simulink model "sschdlexResonantLLCConverterModel"  (R2026a)
settings: Solver=FixedStepDiscrete  StopTime=1e-3
PreLoadFcn:
  | Vdc = 340;
  | Vbus_nominal = 450;
  | Vbus_ripple = 10;
  | busRippleFrequency = 100;
  | Vout_nominal = 54;
  | Pout = 100;
  | Cr = 1.2089e-8;
  | Lr = 1.6226e-4;
  | Lm = 2.3e-3;
  | TR = 4.3269;
  | transformerCoupling = 0.99;
  | Cout = 3.0237e-5;
  | Vf = 0.6;
  | 
  | F_FPGA = 50e6;
  | ts_FPGA_clk  = 1/F_FPGA;
  | ts_cpu= 5e-5;
  | fsw = 100e3;
  | Tbase = ts_FPGA_clk;
  | ts_FPGA_mdl = ts_FPGA_clk;
  | Tdata= ts_FPGA_mdl;
  | 
  | Ts_CAN_Tx = 1e-2;
  | switchType =2 ;
PostLoadFcn:
  | FPGASubsystem_HDLSubsystem_LLCConverter_SolverConfiguration_Gs = Simulink.Parameter;
  | FPGASubsystem_HDLSubsystem_LLCConverter_SolverConfiguration_Gs.Value = 1;
  | FPGASubsystem_HDLSubsystem_LLCConverter_SolverConfiguration_s = Simulink.Parameter;
  | FPGASubsystem_HDLSubsystem_LLCConverter_SolverConfiguration_s.Value = 1;
libraries: SimscapeFPGAHIL_lib x8, ee_lib x6, fl_lib x5, nesl_utility x3, hdlsllib x2
settings Model: DataTypeOverride=Off  Creator=The MathWorks, Inc.  LastModifiedBy=The MathWorks, Inc.
settings OptimizationCC: ConditionallyExecuteInputs=off  InheritOutputTypeSmallerThanSingle=on
settings DebuggingCC: ArtificialAlgebraicLoopMsg=error  SingleTaskRateTransMsg=error
settings HardwareCC: ProdHWDeviceType=ASIC/FPGA->ASIC/FPGA  TargetBitPerLong=64.0  TargetBitPerPointer=64.0  TargetBitPerSizeT=64.0  TargetBitPerPtrDiffT=64.0  TargetLongLongMode=on  TargetIntDivRoundTo=Zero  TargetEndianess=LittleEndian  TargetWordSize=64.0  TargetHWDeviceType=Custom Processor->MATLAB Host Computer  ProdEqTarget=off
settings SimscapeCC: SimscapeNominalValues="[{\"value\":\"1\",\"unit\":\"A\"},{\"value\":\"1\",\"unit\":\"bar\"},{\"value\":\"1\",\"unit\":\"cm^2\"},{\"value\":\"1\",\"unit\":\"cm^3/s\"},{\"value\":\"1\",\"unit\":\"kJ/kg\"},{\"value\":\"1\",\"unit\":\"kW\"},{\"value\":\"1\",\"unit\":\"l\"},{\"value\":\"1\",\"unit\":\"N\"},{\"value\":\"1\",\"unit\":\"N*m\"},{\"value\":\"1\",\"unit\":\"V\"}]"  SimscapeLogType=none  SimscapeLogDataHistory=5000.0

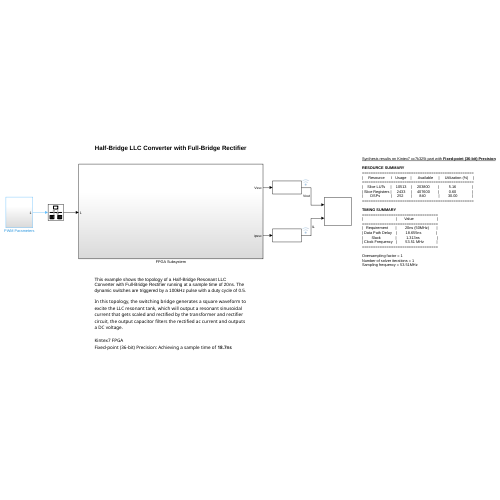
[thumbnail: Simulink's stored preview of the top-level diagram]
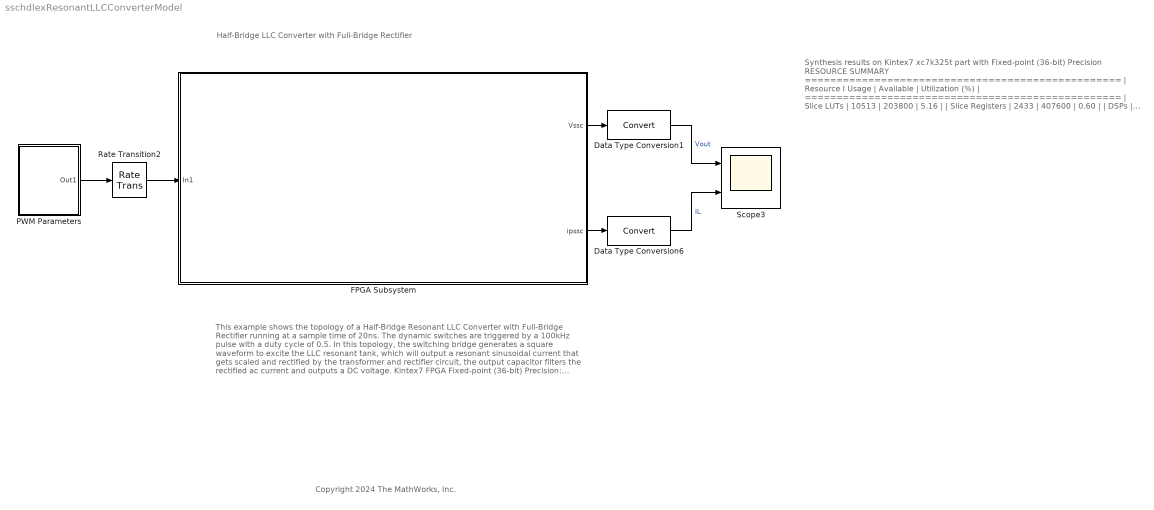
== system sschdlexResonantLLCConverterModel ==
  note: This example shows the topology of a Half-Bridge Resonant LLC Converter with Full-Bridge Rectifier running at a sample time of 20ns. The dynamic switches are triggered by a 100kHz pulse with a duty cycle of 0.5.
      |
      | In this topology, the switching bridge generates a square waveform to excite the LLC resonant tank, which will output a resonant sinusoidal current that gets scaled and rectified by the transformer and rectifier circuit, the output capacitor filters the rectified ac current and outputs a DC voltage.
      |
      | Kintex7 FPGA
      | Fixed-point (36-bit) Precision: Achieving a sample time of 18.7ns
  note: Half-Bridge LLC Converter with Full-Bridge Rectifier
  note: Synthesis results on Kintex7 xc7k325t part with Fixed-point (36-bit) Precision
      |
      | RESOURCE SUMMARY
      | ==================================================
      | | Resource I Usage | Available | Utilization (%) |
      | ==================================================
      | | Slice LUTs | 10513 | 203800 | 5.16 |
      | | Slice Registers | 2433 | 407600 | 0.60 |
      | | DSPs | 252 | 840 | 30.00 |
      | ==================================================
      |
      | TIMING SUMMARY
      | ==================================
      | | | Value |
      | ==================================
      | | Requirement | 20ns (50MHz) |
      | | Data Path Delay | 18.655ns |
      | | Slack | 1.313ns |
      | | Clock Frequency | 53.51 MHz |
      | ==================================
      |
      | Oversampling factor = 1
      | Number of solver iterations = 1
      | Sampling frequency = 53.51MHz
  note: Copyright 2024 The MathWorks, Inc.
  Data Type Conversion1 : DataTypeConversion  SaturateOnIntegerOverflow=off  RndMeth=Floor
  Data Type Conversion6 : DataTypeConversion  SaturateOnIntegerOverflow=off  RndMeth=Floor
  FPGA Subsystem : Subsystem
  PWM Parameters : Subsystem
  Rate Transition2 : RateTransition  OutPortSampleTime=ts_FPGA_clk
  Scope3 : Scope  NumInputPorts=2
      settings: ActiveDisplayYMinimum=-10.52759  ActiveDisplayYMaximum=94.7483
  wires:
  Data Type Conversion1/1 -> Scope3/1  "Vout"
  Data Type Conversion6/1 -> Scope3/2  "IL"
  PWM Parameters/1(Out1) -> Rate Transition2/1
  Rate Transition2/1 -> FPGA Subsystem/1(In1)
  FPGA Subsystem/1(Vssc) -> Data Type Conversion1/1
  FPGA Subsystem/2(ipssc) -> Data Type Conversion6/1

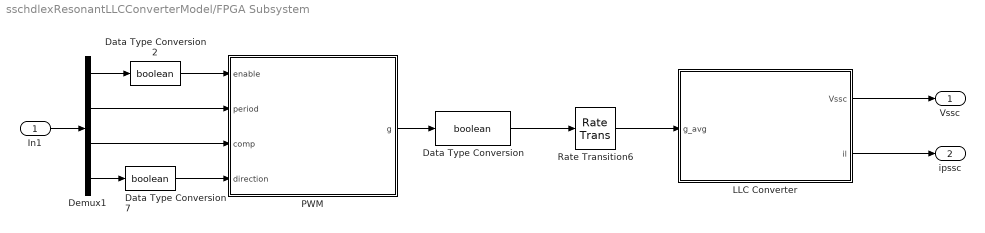
== system sschdlexResonantLLCConverterModel/FPGA Subsystem ==
  In1 : Inport
  Data Type Conversion : DataTypeConversion  OutDataTypeStr=boolean  SaturateOnIntegerOverflow=off  RndMeth=Floor
  Data Type Conversion2 : DataTypeConversion  OutDataTypeStr=boolean  SaturateOnIntegerOverflow=off  RndMeth=Floor
  Data Type Conversion7 : DataTypeConversion  OutDataTypeStr=boolean  SaturateOnIntegerOverflow=off  RndMeth=Floor
  Demux1 : Demux
  LLC Converter : Subsystem
  PWM : Subsystem
  Rate Transition6 : RateTransition
  Vssc : Outport
  ipssc : Outport  Port=2
  wires:
  Demux1/4 -> Data Type Conversion7/1
  Data Type Conversion2/1 -> PWM/1(enable)
  In1/1 -> Demux1/1
  Demux1/1 -> Data Type Conversion2/1
  PWM/1(g) -> Data Type Conversion/1
  Data Type Conversion7/1 -> PWM/4(direction)
  Demux1/3 -> PWM/3(comp)
  Demux1/2 -> PWM/2(period)
  LLC Converter/1(Vssc) -> Vssc/1
  LLC Converter/2(il) -> ipssc/1
  Data Type Conversion/1 -> Rate Transition6/1
  Rate Transition6/1 -> LLC Converter/1(g_avg)

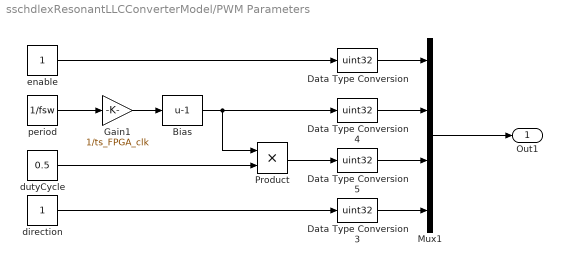
== system sschdlexResonantLLCConverterModel/PWM Parameters ==
  Bias : Bias  Bias=-1  SaturateOnIntegerOverflow=off
  Data Type Conversion{,3..5} (4 alike) : DataTypeConversion  OutDataTypeStr=uint32  SaturateOnIntegerOverflow=off  RndMeth=Floor
  Gain1 : Gain  Gain=1/ts_FPGA_clk
  Mux1 : Mux
  Product : Product
  direction : Constant  SampleTime=ts_cpu
  dutyCycle : Constant  Value=0.5  SampleTime=ts_cpu
  enable : Constant  SampleTime=ts_cpu
  period : Constant  Value=1/fsw  SampleTime=ts_cpu
  Out1 : Outport
  wires:
  Mux1/1 -> Out1/1
  Data Type Conversion/1 -> Mux1/1
  dutyCycle/1 -> Product/2
  Product/1 -> Data Type Conversion5/1
  Gain1/1 -> Bias/1
  Data Type Conversion4/1 -> Mux1/2
  Data Type Conversion3/1 -> Mux1/4
  Data Type Conversion5/1 -> Mux1/3
  period/1 -> Gain1/1
  Bias/1 -> Product/1, Data Type Conversion4/1
  direction/1 -> Data Type Conversion3/1
  enable/1 -> Data Type Conversion/1

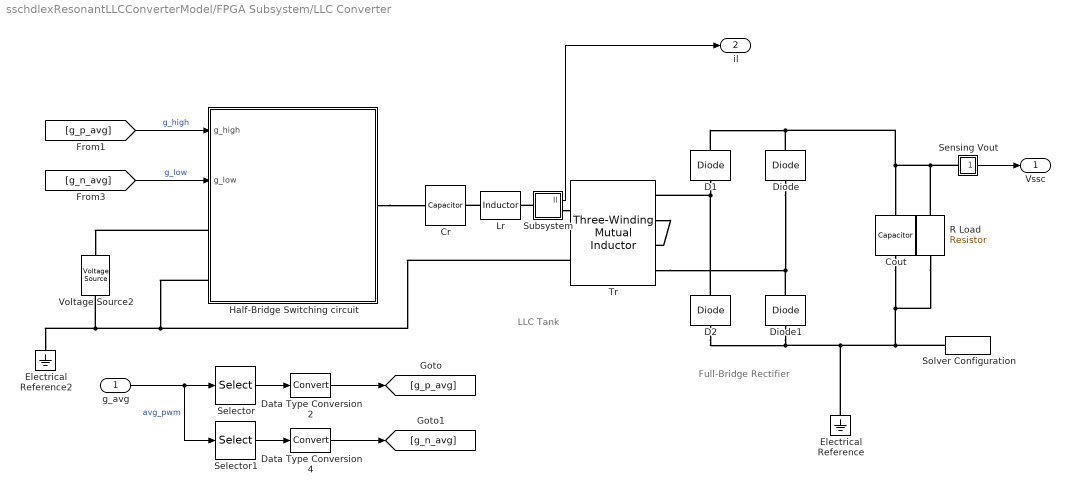
== system sschdlexResonantLLCConverterModel/FPGA Subsystem/LLC Converter ==
  note: LLC Tank
  note: Full-Bridge Rectifier
  g_avg : Inport
  " Half-Bridge Switching circuit" : Subsystem  VariantControl=HB
  Cout : ee_lib/Passive/Capacitor  cap_option=ee.enum.passive.capacitor.capOption.const  c=Cout F  Cvec=[ 1e-5 1e-6 ] F  Vvec=[ 0 10 ] V  CV_table_symmetry=1  f_vec=[1, 10] kHz  DFext_vec=[.8, 1.2]  enable_C_tol=0  averaging_period=0 s  C_tol=5  tol_distribution=1  nSigma=4  r=1e-6 Ohm  g=0 1/Ohm  enable_operating_limits=0  operating_limit_action=2  max_working_voltage_range=[ -25 25 ] V  power_rating=1 W  maxTemperature=85 degC  thermalEnable=false  thermalMass=1 J/K  i_specify=off  i_priority=None  i=0 A  i_nominal_specify=off  i_nominal_value=1  i_nominal_unit=A  v_specify=off  v_priority=None  v=0 V  v_nominal_specify=off  v_nominal_value=1  v_nominal_unit=V  vc_specify=on  vc_priority=High  vc=0 V  vc_nominal_specify=off  vc_nominal_value=1  vc_nominal_unit=V  T_specify=off  T_priority=None  T=298.15 K  T_nominal_specify=off  T_nominal_value=1  T_nominal_unit=K
  Cr : ee_lib/Passive/Capacitor  cap_option=ee.enum.passive.capacitor.capOption.const  c=Cr F  Cvec=[ 1e-5 1e-6 ] F  Vvec=[ 0 10 ] V  CV_table_symmetry=1  f_vec=[1, 10] kHz  DFext_vec=[.8, 1.2]  enable_C_tol=0  averaging_period=0 s  C_tol=5  tol_distribution=1  nSigma=4  r=1e-6 Ohm  g=1e-6 1/Ohm  enable_operating_limits=0  operating_limit_action=2  max_working_voltage_range=[ -25 25 ] V  power_rating=1 W  maxTemperature=85 degC  thermalEnable=false  thermalMass=1 J/K  i_specify=off  i_priority=None  i=0 A  i_nominal_specify=off  i_nominal_value=1  i_nominal_unit=A  v_specify=off  v_priority=None  v=0 V  v_nominal_specify=off  v_nominal_value=1  v_nominal_unit=V  vc_specify=on  vc_priority=High  vc=0 V  vc_nominal_specify=off  vc_nominal_value=1  vc_nominal_unit=V  T_specify=off  T_priority=None  T=298.15 K  T_nominal_specify=off  T_nominal_value=1  T_nominal_unit=K
  D1 : SimscapeFPGAHIL_lib/Dynamic Switch Models/Diode  Vf=0.6  Gs=FPGASubsystem_HDLSubsystem_LLCConverter_SolverConfiguration_Gs  s=FPGASubsystem_HDLSubsystem_LLCConverter_SolverConfiguration_s
  D2 : SimscapeFPGAHIL_lib/Dynamic Switch Models/Diode  Vf=0.6  Gs=FPGASubsystem_HDLSubsystem_LLCConverter_SolverConfiguration_Gs  s=FPGASubsystem_HDLSubsystem_LLCConverter_SolverConfiguration_s
  Data Type Conversion2 : DataTypeConversion  SaturateOnIntegerOverflow=off  RndMeth=Floor
  Data Type Conversion4 : DataTypeConversion  SaturateOnIntegerOverflow=off  RndMeth=Floor
  Diode : SimscapeFPGAHIL_lib/Dynamic Switch Models/Diode  Vf=0.6  Gs=FPGASubsystem_HDLSubsystem_LLCConverter_SolverConfiguration_Gs  s=FPGASubsystem_HDLSubsystem_LLCConverter_SolverConfiguration_s
  Diode1 : SimscapeFPGAHIL_lib/Dynamic Switch Models/Diode  Vf=0.6  Gs=FPGASubsystem_HDLSubsystem_LLCConverter_SolverConfiguration_Gs  s=FPGASubsystem_HDLSubsystem_LLCConverter_SolverConfiguration_s
  Electrical Reference : fl_lib/Electrical/Electrical Elements/Electrical Reference
  Electrical Reference2 : fl_lib/Electrical/Electrical Elements/Electrical Reference
  Lr : ee_lib/Passive/Inductor  l=Lr H  enable_L_tol=0  L_tol=20  tol_distribution=1  nSigma=4  r=0 Ohm  g=1e-9 1/Ohm  enable_operating_limits=0  operating_limit_action=2  max_working_current=1 A  power_rating=1 W  i_L_specify=on  i_L_priority=High  i_L=0 A  i_L_nominal_specify=off  i_L_nominal_value=1  i_L_nominal_unit=A
  R Load : ee_lib/Passive/Resistor  R=Vout_nominal^2/Pout Ohm  enable_R_tol=0  R_tol=5  tol_distribution=1  nSigma=4  enable_operating_limits=0  operating_limit_action=2  power_rating=1 W  max_working_voltage=100 V  noise_mode=0  Tdevice=25 degC  sample_time=0.001 s  repeatability=1  user_seed=0  auto_seed=2715962282  power_derating_T1=70 degC  power_derating_T2=155 degC  operating_temperature_range_vec=[-50, 150] degC  alpha=3.93e-3 1/K  Tmeas=25 degC  thermal_mass=100 J/K  temperature_specify=off  temperature_priority=High  temperature=298.15 K  temperature_nominal_specify=off  temperature_nominal_value=1  temperature_nominal_unit=K
  Selector : Selector  InputPortWidth=2  IndexOptions=Index vector (dialog)  Indices=1  OutputSizes=1
  Selector1 : Selector  InputPortWidth=2  IndexOptions=Index vector (dialog)  Indices=2  OutputSizes=1
  Sensing Vout : Subsystem
      mask Display: disp('v')
  Solver Configuration : nesl_utility/Solver Configuration  PhysicalDomain=network_engine_domain  SubClassName=solver  LeftPortType=input  RightPortType=generic  Tones=[]  Harmonics=[]  SimulateNoise=off  Profile=off  UseLocalSampling=off  EnableSwitchedLinearOptims=on  FrequencyDomain=off  UseCCode=off  RelTol=0.001  AbsTol=1e-06  MinStep=1e-09  ToWorkspace=off  RevertToSquareIcSolve=off  NumHomotopyIterations=100  PhasorMode=off  PhasorModeNumHarmonics=1  ConsistencySolver=NEWTON_FTOL  CanonicalOrdering=UNORDERED  OptimizeIntermediates=UNOPTIMIZED  IndexReductionMethod=DerivativeReplacement  DoDC=off  ResidualTolerance=1e-09  ConsistencyTolSource=GLOBAL  ConsistencyAbsTol=0.001  ConsistencyRelTol=0.001  ConsistencyTolFactor=0.001  UseLocalSolver=on  LocalSolverChoice=NE_BACKWARD_EULER_ADVANCER  ResolveIndetEquations=on  FunctionEvalNumThread=1  LocalSolverSampleTime=ts_FPGA_mdl  DoFixedCost=off  MaxNonlinIter=2  MaxModeIter=2  ComputeImpulses=off  ImpulseIterations=2  LinearAlgebra=auto  LinearAlgebraNumThread=0  EquationFormulation=NE_TIME_EF  DelaysMemoryBudget=1024  AutomaticFiltering=on  FilteringTimeConstant=0.001  PartitionStorageMethod=AS_NEEDED  PartitionMemoryBudget=1024  PartitionMethod=FAST  MultibodyUseLocalSolver=off  MultibodyLocalSolverChoice=ODE1  MultibodyLocalSolverSampleTime=0.001
  Subsystem : Subsystem
  Tr : ee_lib/Passive/Transformers/Three-Winding Mutual Inductor  L1=Lm/transformerCoupling^2 H  L2=Lm/TR^2 H  L3=Lm/TR^2 H  perfectCoupling=false  K12=transformerCoupling  K13=transformerCoupling  K23=transformerCoupling  i1_specify=off  i1_priority=None  i1=0 A  i1_nominal_specify=off  i1_nominal_value=1  i1_nominal_unit=A  i2_specify=on  i2_priority=High  i2=0 A  i2_nominal_specify=off  i2_nominal_value=1  i2_nominal_unit=A  i3_specify=off  i3_priority=None  i3=0 A  i3_nominal_specify=off  i3_nominal_value=1  i3_nominal_unit=A
  Voltage Source2 : ee_lib/Sources/Voltage Source  dc_voltage=Vdc V  ac_voltage=0 V  ac_shift=0 rad  ac_frequency=60 Hz  noise_mode=ee.enum.sources.noise.Disabled  PSD=0 V^2/Hz  sample_time=1e-3 s  repeatability=ee.enum.sources.repeatability.NotRepeatable  user_seed=0  auto_seed=781027040  i_specify=off  i_priority=None  i=0 A  i_nominal_specify=off  i_nominal_value=1  i_nominal_unit=A  v_specify=off  v_priority=None  v=0 V  v_nominal_specify=off  v_nominal_value=1  v_nominal_unit=V
  Vssc : Outport
  il : Outport  Port=2
  wires:
  Data Type Conversion4/1 -> [g_n_avg]
  Data Type Conversion2/1 -> [g_p_avg]
  Selector/1 -> Data Type Conversion2/1
  Selector1/1 -> Data Type Conversion4/1
  g_avg/1 -> Selector/1, Selector1/1  "avg_pwm"
  [g_p_avg] -> " Half-Bridge Switching circuit"/1(g_high)  "g_high"
  [g_n_avg] -> " Half-Bridge Switching circuit"/2(g_low)  "g_low"
  Subsystem/1(Il) -> il/1
  Sensing Vout/1(v) -> Vssc/1
  connections:
  Tr/LConn2 -- " Half-Bridge Switching circuit"/LConn2 -- Electrical Reference2/LConn1 -- Voltage Source2/RConn1
  " Half-Bridge Switching circuit"/LConn1 -- Voltage Source2/LConn1
  Lr/LConn1 -- Cr/RConn1
  Subsystem/RConn1 -- Tr/LConn1
  " Half-Bridge Switching circuit"/RConn1 -- Cr/LConn1
  Subsystem/LConn1 -- Lr/RConn1
  Tr/RConn2 -- Tr/RConn3
  Tr/RConn4 -- Diode/LConn1 -- Diode1/RConn1
  D1/LConn1 -- Tr/RConn1 -- D2/RConn1
  Sensing Vout/LConn1 -- R Load/LConn1 -- D1/RConn1 -- Diode/RConn1 -- Cout/LConn1
  Cout/RConn1 -- Solver Configuration/RConn1 -- Electrical Reference/LConn1 -- D2/LConn1 -- Diode1/LConn1 -- R Load/RConn1

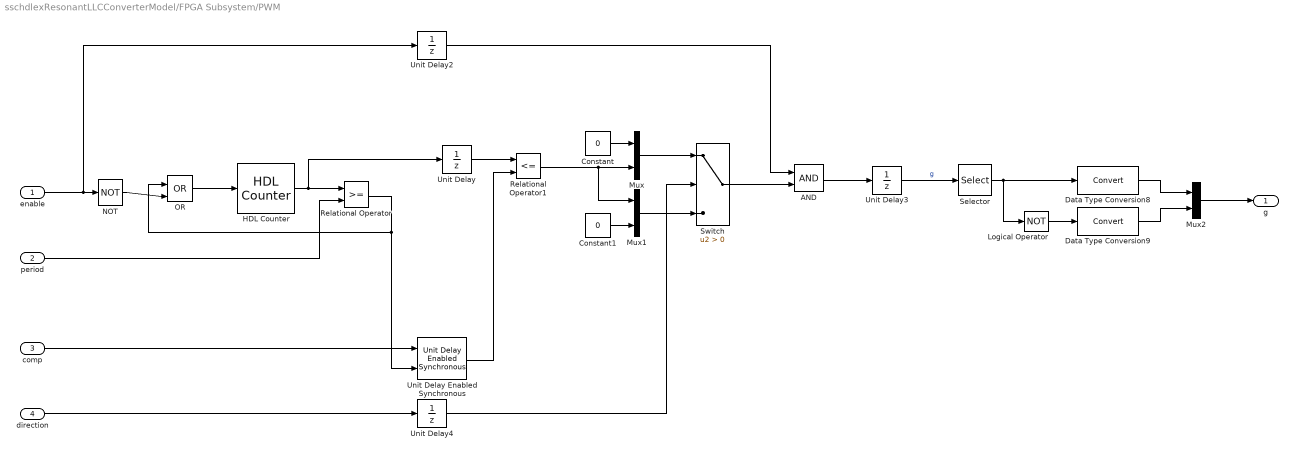
== system sschdlexResonantLLCConverterModel/FPGA Subsystem/PWM ==
  enable : Inport
  period : Inport  Port=2
  comp : Inport  Port=3
  direction : Inport  Port=4
  AND : Logic  AllPortsSameDT=off  OutDataTypeStr=boolean
  Constant : Constant  Value=0  OutDataTypeStr=boolean  SampleTime=-1
  Constant1 : Constant  Value=0  OutDataTypeStr=boolean  SampleTime=-1
  Data Type Conversion8 : DataTypeConversion  SaturateOnIntegerOverflow=off  RndMeth=Floor
  Data Type Conversion9 : DataTypeConversion  SaturateOnIntegerOverflow=off  RndMeth=Floor
  HDL Counter : hdlsllib/Sources/HDL Counter  CountType=Free running  CountInit=0  CountStep=1  CountMax=25  CountFromType=Initial value  CountFrom=0  CountResetPort=on  CountLoadPort=off  CountEnbPort=off  CountDirPort=off  CountHitOutputPort=off  CountDataType=Unsigned  CountWordLen=32  CountFracLen=0  CountSampTime=1
  Logical Operator : Logic  Operator=NOT  AllPortsSameDT=off  OutDataTypeStr=boolean
  Mux : Mux  Inputs=2
  Mux1 : Mux  Inputs=2
  Mux2 : Mux  Inputs=2
  NOT : Logic  Operator=NOT  AllPortsSameDT=off  OutDataTypeStr=boolean
  OR : Logic  Operator=OR  IconShape=distinctive  AllPortsSameDT=off  OutDataTypeStr=boolean
  Relational Operator : RelationalOperator  OutDataTypeStr=boolean  RndMeth=Simplest  InputSameDT=off
  Relational Operator1 : RelationalOperator  Operator=<=  OutDataTypeStr=boolean  RndMeth=Simplest  InputSameDT=off
  Selector : Selector  InputPortWidth=2  IndexOptions=Index vector (dialog)  Indices=[2]  OutputSizes=1
  Switch : Switch  Criteria=u2 > Threshold  SaturateOnIntegerOverflow=off  InputSameDT=off
  Unit Delay{,2..4} (4 alike) : UnitDelay  SampleTime=-1
  Unit Delay Enabled Synchronous : hdlsllib/Discrete/Unit Delay Enabled Synchronous  InitialCondition=0.0  SampleTime=-1
  g : Outport
  wires:
  comp/1 -> Unit Delay Enabled Synchronous/1
  Unit Delay3/1 -> Selector/1  "g"
  period/1 -> Relational Operator/2
  Switch/1 -> AND/2
  Unit Delay/1 -> Relational Operator1/1
  direction/1 -> Unit Delay4/1
  AND/1 -> Unit Delay3/1
  Mux/1 -> Switch/1
  Constant1/1 -> Mux1/2
  Unit Delay2/1 -> AND/1
  Mux1/1 -> Switch/3
  Constant/1 -> Mux/1
  Relational Operator/1 -> OR/1, Unit Delay Enabled Synchronous/2
  enable/1 -> NOT/1, Unit Delay2/1
  HDL Counter/1 -> Relational Operator/1, Unit Delay/1
  Unit Delay4/1 -> Switch/2
  Unit Delay Enabled Synchronous/1 -> Relational Operator1/2
  OR/1 -> HDL Counter/1
  Relational Operator1/1 -> Mux/2, Mux1/1
  NOT/1 -> OR/2
  Data Type Conversion9/1 -> Mux2/2
  Data Type Conversion8/1 -> Mux2/1
  Logical Operator/1 -> Data Type Conversion9/1
  Selector/1 -> Logical Operator/1, Data Type Conversion8/1
  Mux2/1 -> g/1

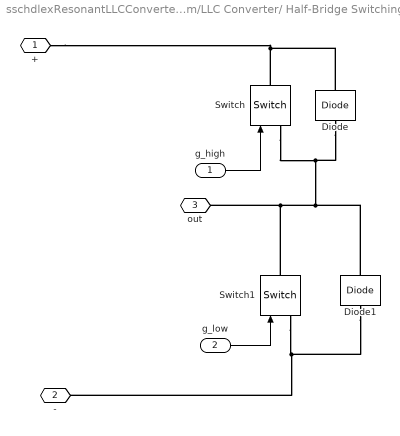
== system sschdlexResonantLLCConverterModel/FPGA Subsystem/LLC Converter/ Half-Bridge Switching circuit ==
  g_high : Inport
  g_low : Inport  Port=2
  Diode : SimscapeFPGAHIL_lib/Dynamic Switch Models/Diode  Vf=0.6  Gs=FPGASubsystem_HDLSubsystem_LLCConverter_SolverConfiguration_Gs  s=FPGASubsystem_HDLSubsystem_LLCConverter_SolverConfiguration_s
  Diode1 : SimscapeFPGAHIL_lib/Dynamic Switch Models/Diode  Vf=0.6  Gs=FPGASubsystem_HDLSubsystem_LLCConverter_SolverConfiguration_Gs  s=FPGASubsystem_HDLSubsystem_LLCConverter_SolverConfiguration_s
  Switch : SimscapeFPGAHIL_lib/Dynamic Switch Models/Switch  device_type=Switch  threshold=0.5  Gs=FPGASubsystem_HDLSubsystem_LLCConverter_SolverConfiguration_Gs  s=FPGASubsystem_HDLSubsystem_LLCConverter_SolverConfiguration_s
  Switch1 : SimscapeFPGAHIL_lib/Dynamic Switch Models/Switch  device_type=Switch  threshold=0.5  Gs=FPGASubsystem_HDLSubsystem_LLCConverter_SolverConfiguration_Gs  s=FPGASubsystem_HDLSubsystem_LLCConverter_SolverConfiguration_s
  + : PMIOPort  Side=Left
  - : PMIOPort  Port=2  Side=Left
  out : PMIOPort  Port=3  Side=Right
  wires:
  g_high/1 -> Switch/1
  g_low/1 -> Switch1/1
  connections:
  +/RConn1 -- Diode/RConn1 -- Switch/RConn1
  Diode1/LConn1 -- Switch1/LConn1 -- -/RConn1
  Diode/LConn1 -- Switch/LConn1 -- out/RConn1 -- Switch1/RConn1 -- Diode1/RConn1

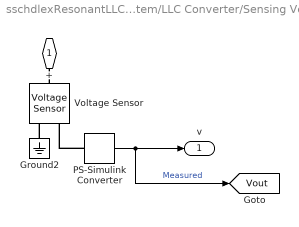
== system sschdlexResonantLLCConverterModel/FPGA Subsystem/LLC Converter/Sensing Vout ==
  Ground2 : fl_lib/Electrical/Electrical Elements/Electrical Reference
  PS-Simulink Converter : nesl_utility/PS-Simulink Converter  PhysicalDomain=network_engine_domain  SubClassName=ps_output  LeftPortType=input  RightPortType=output  PseudoPeriodic=off  Frequencies=[]  VectorFormat=1-D array  Unit=1  AffineConversion=off
  Voltage Sensor : fl_lib/Electrical/Electrical Sensors/Voltage Sensor
  + : PMIOPort  Side=Left
  v : Outport  VectorParamsAs1DForOutWhenUnconnected=off
  tag scope: Vout=global
  wires:
  PS-Simulink Converter/1 -> [Vout], v/1  "Measured"
  connections:
  PS-Simulink Converter/LConn1 -- Voltage Sensor/RConn1
  Ground2/LConn1 -- Voltage Sensor/RConn2
  Voltage Sensor/LConn1 -- +/RConn1

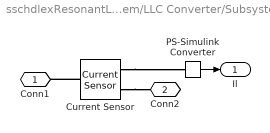
== system sschdlexResonantLLCConverterModel/FPGA Subsystem/LLC Converter/Subsystem ==
  Current Sensor : fl_lib/Electrical/Electrical Sensors/Current Sensor
  PS-Simulink Converter : nesl_utility/PS-Simulink Converter  PhysicalDomain=network_engine_domain  SubClassName=ps_output  LeftPortType=input  RightPortType=output  PseudoPeriodic=off  Frequencies=[]  VectorFormat=inherit  Unit=inherit  AffineConversion=off
  Conn1 : PMIOPort  Side=Left
  Conn2 : PMIOPort  Port=2  Side=Right
  Il : Outport
  wires:
  PS-Simulink Converter/1 -> Il/1
  connections:
  Current Sensor/RConn1 -- PS-Simulink Converter/LConn1
  Current Sensor/RConn2 -- Conn2/RConn1
  Current Sensor/LConn1 -- Conn1/RConn1
